simulink model "dpsim_sg_3ph_reference"  (R2025a)
settings: Solver=ode15s  StartTime=0  StopTime=4  MaxStep=5.0000000000000002e-05  RelTol=1e-7  AbsTol=1e-9
settings Model: Creator=matthiasmees  LastModifiedBy=matthiasmees

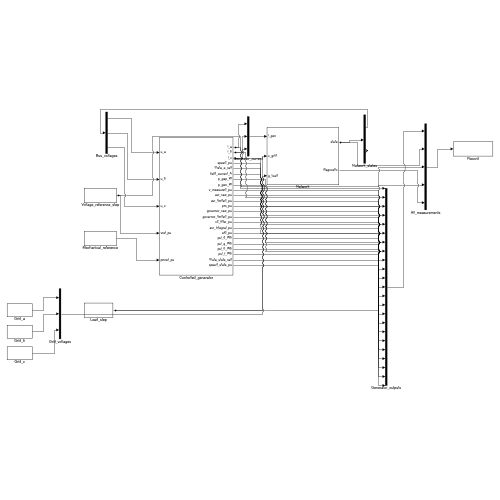
[thumbnail: Simulink's stored preview of the top-level diagram]
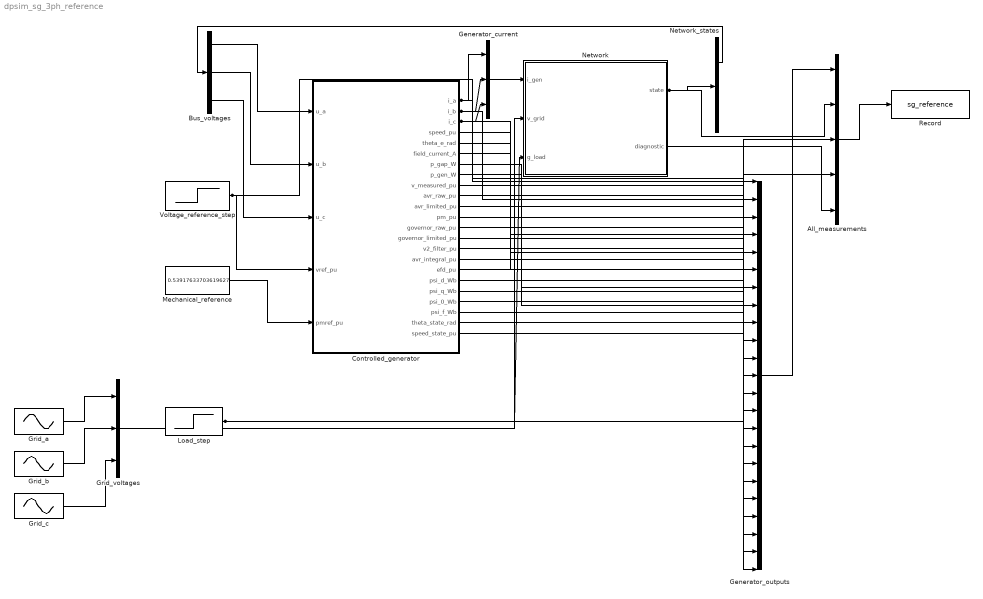
== system dpsim_sg_3ph_reference ==
  All_measurements : Mux  Inputs=5
  Bus_voltages : Demux  Outputs=3
  Controlled_generator : Subsystem
  Generator_current : Mux  Inputs=3
  Generator_outputs : Mux  Inputs=23
  Grid_a : Sin  Amplitude=325.26911934581187  Frequency=314.15926535897933  Phase=1.5707963267948966  SampleTime=0
  Grid_b : Sin  Amplitude=325.26911934581187  Frequency=314.15926535897933  Phase=-0.5235987755982987  SampleTime=0
  Grid_c : Sin  Amplitude=325.26911934581187  Frequency=314.15926535897933  Phase=3.6651914291880918  SampleTime=0
  Grid_voltages : Mux  Inputs=3
  Load_step : Step  Before=0.03780718336483932  After=0.075614366729678639  SampleTime=0
  Mechanical_reference : Constant  Value=0.53917633703619627
  Network : Subsystem
  Network_states : Demux  Outputs=[3 3]
  Record : ToWorkspace  VariableName=sg_reference  SaveFormat=Timeseries  SampleTime=-1
  Voltage_reference_step : Step  Time=2  Before=1  After=1.02  SampleTime=0
  wires:
  Network/1(state) -> Network_states/1, All_measurements/2
  Network_states/1 -> Bus_voltages/1
  Bus_voltages/1 -> Controlled_generator/1(u_a)
  Controlled_generator/1(i_a) -> Generator_current/1, Generator_outputs/1
  Bus_voltages/2 -> Controlled_generator/2(u_b)
  Controlled_generator/2(i_b) -> Generator_current/2, Generator_outputs/2
  Bus_voltages/3 -> Controlled_generator/3(u_c)
  Controlled_generator/3(i_c) -> Generator_current/3, Generator_outputs/3
  Generator_current/1 -> Network/1(i_gen)
  Grid_a/1 -> Grid_voltages/1
  Grid_b/1 -> Grid_voltages/2
  Grid_c/1 -> Grid_voltages/3
  Grid_voltages/1 -> Network/2(v_grid)
  Load_step/1 -> Network/3(g_load), All_measurements/3
  Voltage_reference_step/1 -> Controlled_generator/4(vref_pu), All_measurements/4
  Mechanical_reference/1 -> Controlled_generator/5(pmref_pu)
  Controlled_generator/4(speed_pu) -> Generator_outputs/4
  Controlled_generator/5(theta_e_rad) -> Generator_outputs/5
  Controlled_generator/6(field_current_A) -> Generator_outputs/6
  Controlled_generator/7(p_gap_W) -> Generator_outputs/7
  Controlled_generator/8(p_gen_W) -> Generator_outputs/8
  Controlled_generator/9(v_measured_pu) -> Generator_outputs/9
  Controlled_generator/10(avr_raw_pu) -> Generator_outputs/10
  Controlled_generator/11(avr_limited_pu) -> Generator_outputs/11
  Controlled_generator/12(pm_pu) -> Generator_outputs/12
  Controlled_generator/13(governor_raw_pu) -> Generator_outputs/13
  Controlled_generator/14(governor_limited_pu) -> Generator_outputs/14
  Controlled_generator/15(v2_filter_pu) -> Generator_outputs/15
  Controlled_generator/16(avr_integral_pu) -> Generator_outputs/16
  Controlled_generator/17(efd_pu) -> Generator_outputs/17
  Controlled_generator/18(psi_d_Wb) -> Generator_outputs/18
  Controlled_generator/19(psi_q_Wb) -> Generator_outputs/19
  Controlled_generator/20(psi_0_Wb) -> Generator_outputs/20
  Controlled_generator/21(psi_f_Wb) -> Generator_outputs/21
  Controlled_generator/22(theta_state_rad) -> Generator_outputs/22
  Controlled_generator/23(speed_state_pu) -> Generator_outputs/23
  Generator_outputs/1 -> All_measurements/1
  Network/2(diagnostic) -> All_measurements/5
  All_measurements/1 -> Record/1

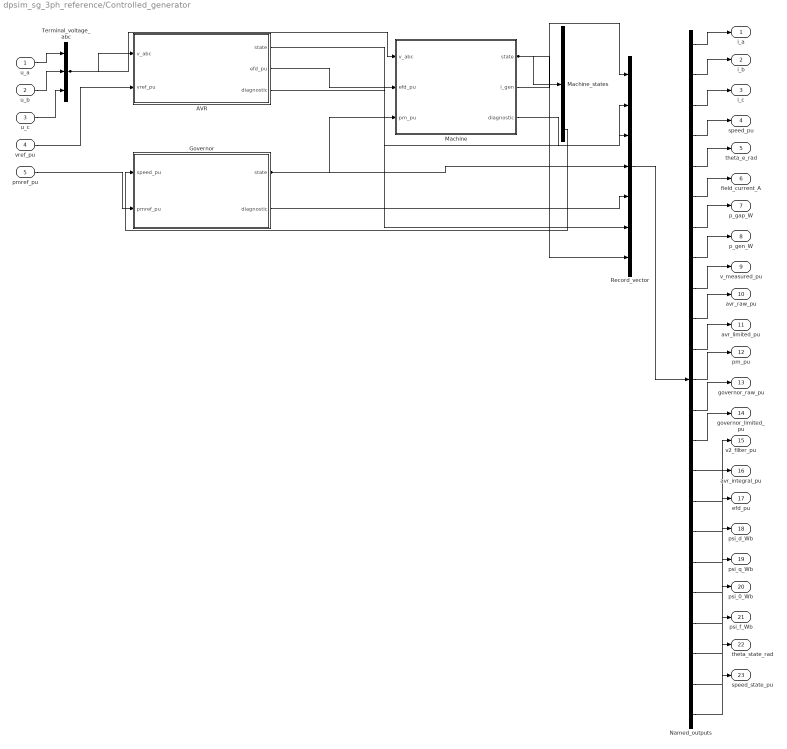
== system dpsim_sg_3ph_reference/Controlled_generator ==
  u_a : Inport  OutDataTypeStr=double  PortDimensions=1  SampleTime=0
  u_b : Inport  Port=2  OutDataTypeStr=double  PortDimensions=1  SampleTime=0
  u_c : Inport  Port=3  OutDataTypeStr=double  PortDimensions=1  SampleTime=0
  vref_pu : Inport  Port=4  OutDataTypeStr=double  PortDimensions=1  SampleTime=0
  pmref_pu : Inport  Port=5  OutDataTypeStr=double  PortDimensions=1  SampleTime=0
  AVR : Subsystem
  Governor : Subsystem
  Machine : Subsystem
  Machine_states : Demux  Outputs=6
  Named_outputs : Demux  Outputs=23
  Record_vector : Mux  Inputs=7
  Terminal_voltage_abc : Mux  Inputs=3
  i_a : Outport
  i_b : Outport  Port=2
  i_c : Outport  Port=3
  speed_pu : Outport  Port=4
  theta_e_rad : Outport  Port=5
  field_current_A : Outport  Port=6
  p_gap_W : Outport  Port=7
  p_gen_W : Outport  Port=8
  v_measured_pu : Outport  Port=9
  avr_raw_pu : Outport  Port=10
  avr_limited_pu : Outport  Port=11
  pm_pu : Outport  Port=12
  governor_raw_pu : Outport  Port=13
  governor_limited_pu : Outport  Port=14
  v2_filter_pu : Outport  Port=15
  avr_integral_pu : Outport  Port=16
  efd_pu : Outport  Port=17
  psi_d_Wb : Outport  Port=18
  psi_q_Wb : Outport  Port=19
  psi_0_Wb : Outport  Port=20
  psi_f_Wb : Outport  Port=21
  theta_state_rad : Outport  Port=22
  speed_state_pu : Outport  Port=23
  wires:
  u_a/1 -> Terminal_voltage_abc/1
  u_b/1 -> Terminal_voltage_abc/2
  u_c/1 -> Terminal_voltage_abc/3
  Terminal_voltage_abc/1 -> AVR/1(v_abc), Machine/1(v_abc)
  vref_pu/1 -> AVR/2(vref_pu)
  AVR/2(efd_pu) -> Machine/2(efd_pu)
  Governor/1(state) -> Record_vector/4, Machine/3(pm_pu)
  Machine/1(state) -> Record_vector/7, Machine_states/1
  Machine_states/6 -> Governor/1(speed_pu)
  pmref_pu/1 -> Governor/2(pmref_pu)
  Machine/2(i_gen) -> Record_vector/1
  Machine/3(diagnostic) -> Record_vector/2
  AVR/3(diagnostic) -> Record_vector/3
  Governor/2(diagnostic) -> Record_vector/5
  AVR/1(state) -> Record_vector/6
  Record_vector/1 -> Named_outputs/1
  Named_outputs/1 -> i_a/1
  Named_outputs/2 -> i_b/1
  Named_outputs/3 -> i_c/1
  Named_outputs/4 -> speed_pu/1
  Named_outputs/5 -> theta_e_rad/1
  Named_outputs/6 -> field_current_A/1
  Named_outputs/7 -> p_gap_W/1
  Named_outputs/8 -> p_gen_W/1
  Named_outputs/9 -> v_measured_pu/1
  Named_outputs/10 -> avr_raw_pu/1
  Named_outputs/11 -> avr_limited_pu/1
  Named_outputs/12 -> pm_pu/1
  Named_outputs/13 -> governor_raw_pu/1
  Named_outputs/14 -> governor_limited_pu/1
  Named_outputs/15 -> v2_filter_pu/1
  Named_outputs/16 -> avr_integral_pu/1
  Named_outputs/17 -> efd_pu/1
  Named_outputs/18 -> psi_d_Wb/1
  Named_outputs/19 -> psi_q_Wb/1
  Named_outputs/20 -> psi_0_Wb/1
  Named_outputs/21 -> psi_f_Wb/1
  Named_outputs/22 -> theta_state_rad/1
  Named_outputs/23 -> speed_state_pu/1

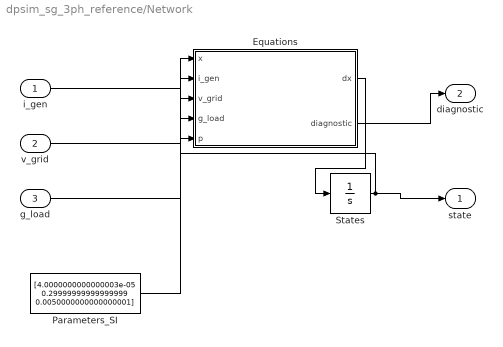
== system dpsim_sg_3ph_reference/Network ==
  i_gen : Inport
  v_grid : Inport  Port=2
  g_load : Inport  Port=3
  Equations : MATLAB Function  TreatAsAtomicUnit=on
  Parameters_SI : Constant  Value=[4.0000000000000003e-05 0.29999999999999999 0.0050000000000000001]
  States : Integrator  InitialCondition=[325.20091289985112;-156.83203493034051;-168.36887796951044;4.0831676149501721;-1.3286291356711253;-2.7545384792790446]
  state : Outport
  diagnostic : Outport  Port=2
  wires:
  States/1 -> Equations/1(x), state/1
  i_gen/1 -> Equations/2(i_gen)
  v_grid/1 -> Equations/3(v_grid)
  g_load/1 -> Equations/4(g_load)
  Parameters_SI/1 -> Equations/5(p)
  Equations/1(dx) -> States/1
  Equations/2(diagnostic) -> diagnostic/1

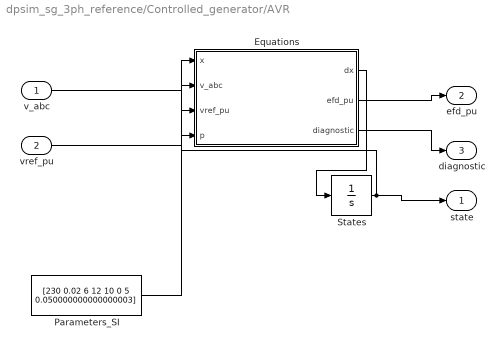
== system dpsim_sg_3ph_reference/Controlled_generator/AVR ==
  v_abc : Inport
  vref_pu : Inport  Port=2
  Equations : MATLAB Function  TreatAsAtomicUnit=on
  Parameters_SI : Constant  Value=[230 0.02 6 12 10 0 5 0.050000000000000003]
  States : Integrator  InitialCondition=[1;1.1797929749436427;1.1797929749436427]
  state : Outport
  efd_pu : Outport  Port=2
  diagnostic : Outport  Port=3
  wires:
  Equations/3(diagnostic) -> diagnostic/1
  Equations/2(efd_pu) -> efd_pu/1
  Equations/1(dx) -> States/1
  Parameters_SI/1 -> Equations/4(p)
  vref_pu/1 -> Equations/3(vref_pu)
  v_abc/1 -> Equations/2(v_abc)
  States/1 -> state/1, Equations/1(x)

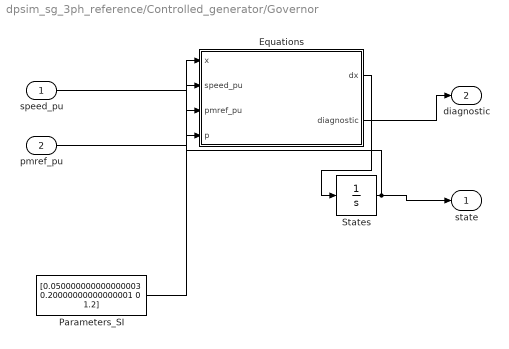
== system dpsim_sg_3ph_reference/Controlled_generator/Governor ==
  speed_pu : Inport
  pmref_pu : Inport  Port=2
  Equations : MATLAB Function  TreatAsAtomicUnit=on
  Parameters_SI : Constant  Value=[0.050000000000000003 0.20000000000000001 0 1.2]
  States : Integrator  InitialCondition=0.53917633703619627
  state : Outport
  diagnostic : Outport  Port=2
  wires:
  Equations/2(diagnostic) -> diagnostic/1
  Equations/1(dx) -> States/1
  Parameters_SI/1 -> Equations/4(p)
  pmref_pu/1 -> Equations/3(pmref_pu)
  speed_pu/1 -> Equations/2(speed_pu)
  States/1 -> state/1, Equations/1(x)

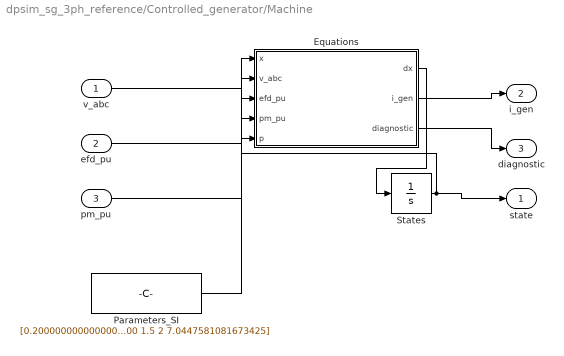
== system dpsim_sg_3ph_reference/Controlled_generator/Machine ==
  v_abc : Inport
  efd_pu : Inport  Port=2
  pm_pu : Inport  Port=3
  Equations : MATLAB Function  TreatAsAtomicUnit=on
  Parameters_SI : Constant  Value=[0.20000000000000001 0.059999999999999998 0.044999999999999998 0.01 1.5 0.27000000000000002 1.5 314.15926535897933 15000 1.5 2 7.0447581081673425]
  States : Integrator  InitialCondition=[0.95730040521907422;-0.8509662175152457;0;5.887009487462521;-0.82071744650734413;1]
  state : Outport
  i_gen : Outport  Port=2
  diagnostic : Outport  Port=3
  wires:
  Equations/3(diagnostic) -> diagnostic/1
  Equations/2(i_gen) -> i_gen/1
  Equations/1(dx) -> States/1
  Parameters_SI/1 -> Equations/5(p)
  pm_pu/1 -> Equations/4(pm_pu)
  efd_pu/1 -> Equations/3(efd_pu)
  v_abc/1 -> Equations/2(v_abc)
  States/1 -> state/1, Equations/1(x)

== matlab function dpsim_sg_3ph_reference/Controlled_generator/AVR/Equations ==
  data: x input; dx output; v_abc input; vref_pu input; p input; efd_pu output; diagnostic output
function [dx, efd_pu, diagnostic] = sg_avr_rhs(x, v_abc, vref_pu, p)
%#codegen
% x = [filtered squared RMS voltage pu; PI integrator; exciter voltage pu].
% p = [VphaseBase Tmeasure Kp Ki Kaw EfdMin EfdMax Texciter].
v2 = (v_abc.'*v_abc)/(3*p(1)^2);
vmeasure = sqrt(max(x(1),1e-12));
error = vref_pu-vmeasure;
raw = x(2)+p(3)*error;
limited = min(max(raw,p(6)),p(7));
dx = [(v2-x(1))/p(2); p(4)*error+p(5)*(limited-raw); ...
      (limited-x(3))/p(8)];
efd_pu=x(3);
diagnostic=[vmeasure; raw; limited];
end

== matlab function dpsim_sg_3ph_reference/Controlled_generator/Machine/Equations ==
  data: x input; dx output; v_abc input; efd_pu input; pm_pu input; p input; i_gen output; diagnostic output
function [dx, i_gen, diagnostic] = sg_machine_rhs(x, v_abc, efd_pu, pm_pu, p)
%#codegen
% Power-invariant Park coordinates, passive stator current INTO machine.
% x = [psi_d; psi_q; psi_0; psi_f; theta_e; speed_pu].
% p = [Rs Ld Lq L0 Lf M Rf wb Sbase H D Vfbase].
Rs=p(1); Ld=p(2); Lq=p(3); L0=p(4); Lf=p(5); M=p(6);
Rf=p(7); wb=p(8); Sbase=p(9); H=p(10); D=p(11); Vfbase=p(12);
a = x(5) + [0; -2*pi/3; 2*pi/3];
T = sqrt(2/3)*[cos(a).'; -sin(a).'; ones(1,3)/sqrt(2)];
v = T*v_abc;
% Symmetric flux/current matrix: magnetic energy is positive definite.
id = (Lf*x(1)-M*x(4))/(Ld*Lf-M*M);
ifield = (Ld*x(4)-M*x(1))/(Ld*Lf-M*M);
iq=x(2)/Lq; i0=x(3)/L0;
i_passive = [id; iq; i0];
i_gen = -T.'*i_passive; % positive OUT of generator, INTO bus
we = wb*x(6);
% For a power-invariant transform, no 3/2 factor appears in power/torque.
p_gap = -we*(x(1)*iq-x(2)*id);
dx = zeros(6,1);
dx(1) = v(1)-Rs*id+we*x(2);
dx(2) = v(2)-Rs*iq-we*x(1);
dx(3) = v(3)-Rs*i0;
dx(4) = Vfbase*efd_pu-Rf*ifield;
dx(5) = we;
% Kinetic energy = H*Sbase*speed_pu^2; D is damping in power per pu speed.
dx(6) = (pm_pu-p_gap/Sbase-D*(x(6)-1))/(2*H*x(6));
diagnostic = [x(6); x(5); ifield; p_gap; v_abc.'*i_gen];
end

== matlab function dpsim_sg_3ph_reference/Controlled_generator/Governor/Equations ==
  data: x input; dx output; speed_pu input; pmref_pu input; p input; diagnostic output
function [dx, diagnostic] = sg_governor_rhs(x, speed_pu, pmref_pu, p)
%#codegen
% One first-order prime mover with droop, not a turbine-specific model.
% p = [droop Tgovernor Pmin Pmax].
raw = pmref_pu+(1-speed_pu)/p(1);
limited = min(max(raw,p(3)),p(4));
dx = (limited-x)/p(2);
diagnostic=[raw; limited];
end

== matlab function dpsim_sg_3ph_reference/Network/Equations ==
  data: x input; dx output; i_gen input; v_grid input; g_load input; p input; diagnostic output
function [dx, diagnostic] = sg_network_rhs(x, i_gen, v_grid, g_load, p)
%#codegen
% x = [v_bus_abc; i_line_abc], line current positive from bus to grid.
% p = [Cbus Rline Lline], load conductance in S PER PHASE.
v=x(1:3); iline=x(4:6);
i_load=g_load*v;
dx=[(i_gen-iline-i_load)/p(1); (v-v_grid-p(2)*iline)/p(3)];
diagnostic=[v.'*i_load; v.'*iline; p(2)*(iline.'*iline)];
end
